simulink model "TorqueTest"  (R2026a)
settings: Solver=FixedStepAuto  StopTime=15  FixedStep=0.001  MinStep=1e-4
model workspace (MATLAB code in the model file):
  | K_d_1 = 0;
  | omegaFilter = 100;
  | 
  | 
  | % Motor parmeters
  | Km = 0.5;
  | 
  | % Gear ratio
  | i = 20;
  | 
  | %
  | IMax = 16;
  | IMin = - IMax;
undefined symbols (not defined in the file or in its folder): X, Y, Z
libraries: sm_lib x26, nesl_utility x16, slpidlib x1
settings Model: Creator=Bruker  LastModifiedBy=Bruker

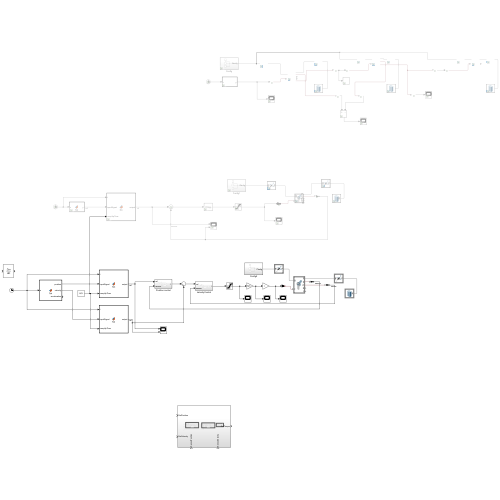
[thumbnail: Simulink's stored preview of the top-level diagram]
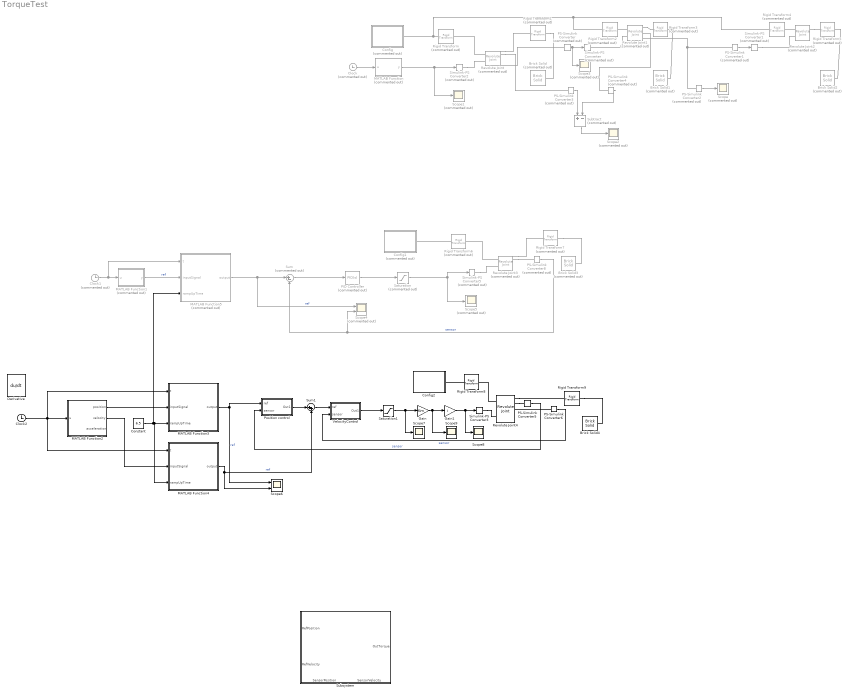
== system TorqueTest ==
  Brick Solid{,1..3} (4 alike) : sm_lib/Body Elements/Brick Solid  Commented=on  BrickDimensions=[1 0.1 0.1]  BrickDimensionsUnits=m  ExportEntireGeometry=off  InertiaType=CalculateFromGeometry  BasedOnType=Density  Density=1000  DensityUnits=kg/m^3  Mass=1  MassUnits=kg  CenterOfMass=[0 0 0]  CenterOfMassUnits=m  MomentsOfInertia=[1 1 1]  MomentsOfInertiaUnits=kg*m^2  ProductsOfInertia=[0 0 0]  ProductsOfInertiaUnits=kg*m^2  GraphicType=FromGeometry  MarkerShape=Sphere  MarkerSize=10  GraphicVisPropType=SimpleVisualProperties  GraphicDiffuseColor=[0.5 0.5 0.5]  GraphicOpacity=1  GraphicSpecularColor=[0.5 0.5 0.5 1.0]  GraphicAmbientColor=[0.15 0.15 0.15 1.0]  GraphicEmissiveColor=[0.0 0.0 0.0 1.0]  GraphicShininess=75  DoExposeReferenceFrame=on  SerializedFrames=<Frames/>
  Brick Solid4 : sm_lib/Body Elements/Brick Solid  BrickDimensions=[1 0.1 0.1]  BrickDimensionsUnits=m  ExportEntireGeometry=off  InertiaType=CalculateFromGeometry  BasedOnType=Density  Density=1000  DensityUnits=kg/m^3  Mass=1  MassUnits=kg  CenterOfMass=[0 0 0]  CenterOfMassUnits=m  MomentsOfInertia=[1 1 1]  MomentsOfInertiaUnits=kg*m^2  ProductsOfInertia=[0 0 0]  ProductsOfInertiaUnits=kg*m^2  GraphicType=FromGeometry  MarkerShape=Sphere  MarkerSize=10  GraphicVisPropType=SimpleVisualProperties  GraphicDiffuseColor=[0 0.3333 1]  GraphicOpacity=1  GraphicSpecularColor=[0.5 0.5 0.5 1.0]  GraphicAmbientColor=[0.15 0.15 0.15 1.0]  GraphicEmissiveColor=[0.0 0.0 0.0 1.0]  GraphicShininess=75  DoExposeReferenceFrame=on  SerializedFrames=<Frames/>
  Clock : Clock  Commented=on
  Clock1 : Clock  Commented=on
  Clock2 : Clock
  Config : Subsystem  Commented=on
  Config1 : Subsystem  Commented=on
  Config2 : Subsystem
  Constant : Constant  Value=6.5
  Derivative : Derivative
  Gain : Gain  Gain=Km
  Gain1 : Gain  Gain=i
  MATLAB Function : MATLAB Function  Commented=on  TreatAsAtomicUnit=on
  MATLAB Function1 : MATLAB Function  Commented=on  TreatAsAtomicUnit=on
  MATLAB Function2 : MATLAB Function  TreatAsAtomicUnit=on
  MATLAB Function3 : MATLAB Function  TreatAsAtomicUnit=on
  MATLAB Function4 : MATLAB Function  TreatAsAtomicUnit=on
  MATLAB Function5 : MATLAB Function  Commented=on  TreatAsAtomicUnit=on
  PID Controller : slpidlib/PID Controller  Commented=on  Controller=PID  Form=Parallel  TimeDomain=Continuous-time  UseExternalTs=off  SampleTime=-1  IntegratorMethod=Forward Euler  FilterMethod=Forward Euler  ControllerParametersSource=internal  P=750  I=0  UseKiTs=off  D=10  UseExternalDerivativeSource=off  N=100  UseFilter=on  TunerSelectOption=Transfer Function Based (PID Tuner App)  InitialConditionSource=internal  InitialConditionForIntegrator=0  InitialConditionForFilter=0  DifferentiatorICPrevScaledInput=0  ExternalReset=none  TrackingMode=off  Kt=1  LimitOutput=off  SatLimitsSource=internal  UpperSaturationLimit=inf  LowerSaturationLimit=-inf  LinearizeAsGain=on  AntiWindupMode=none  Kb=1  LimitIntegrator=off  UpperIntegratorSaturationLimit=inf  LowerIntegratorSaturationLimit=-inf  POutMin=[]  POutMax=[]  IOutMin=[]  IOutMax=[]  DOutMin=[]  DOutMax=[]  NOutMin=[]  NOutMax=[]  SumOutMin=[]  SumOutMax=[]  SaturationOutMin=[]  SaturationOutMax=[]  PParamMin=[]  PParamMax=[]  IParamMin=[]  IParamMax=[]  DParamMin=[]  DParamMax=[]  NParamMin=[]  NParamMax=[]  KbParamMin=[]  KbParamMax=[]  KtParamMin=[]  KtParamMax=[]  KbOutMin=[]  KbOutMax=[]  KtOutMin=[]  KtOutMax=[]  IntegratorOutMin=[]  IntegratorOutMax=[]  FilterOutMin=[]  FilterOutMax=[]  SumI1OutMin=[]  SumI1OutMax=[]  SumI2OutMin=[]  SumI2OutMax=[]  SumI3OutMin=[]  SumI3OutMax=[]  SumI4OutMin=[]  SumI4OutMax=[]  SumDOutMin=[]  SumDOutMax=[]  DifferentiatorOutMin=[]  DifferentiatorOutMax=[]  FilterDiffOutCoefMin=[]  FilterDiffOutCoefMax=[]  ReciprocalOutMin=[]  ReciprocalOutMax=[]  SumDenOutMin=[]  SumDenOutMax=[]  SumNumOutMin=[]  SumNumOutMax=[]  DivideOutMin=[]  DivideOutMax=[]  UdiffTsProdOutMin=[]  UdiffTsProdOutMax=[]  NTsProdOutMin=[]  NTsProdOutMax=[]  UintegralTsProdOutMin=[]  UintegralTsProdOutMax=[]  UngainTsProdOutMin=[]  UngainTsProdOutMax=[]  ClampingZeroOutDataTypeStr=Inherit: Inherit via back propagation  ClampingZeroOutMin=[]  ClampingZeroOutMax=[]  FilterDenConstantOutDataTypeStr=Inherit: Inherit via back propagation  FilterDenConstantOutMin=[]  FilterDenConstantOutMax=[]  PCopyOutDataTypeStr=Inherit: Inherit via back propagation  PCopyOutMin=[]  PCopyOutMax=[]  NCopyOutDataTypeStr=Inherit: Inherit via back propagation  NCopyOutMin=[]  NCopyOutMax=[]  IntegratorContinuousStateAttributes=''  IntegratorStateMustResolveToSignalObject=off  IntegratorRTWStateStorageClass=Auto  FilterContinuousStateAttributes=''  FilterStateMustResolveToSignalObject=off  FilterRTWStateStorageClass=Auto  ParallelPVariant=InternalParameters  IdealPVariant=Disabled  IVariant=InternalParameters  DVariant=InternalParameters  IntegratorVariant=Continuous  SatVariant=Disabled  AWVariant=Passthrough  PCopyVariant=Disabled  TRVariant=Disabled  FdbkBlocksVariant=Forward  IdealPFdbkVariant=Disabled  SatFdbkVariant=Disabled  DerivativeFilterVariant=ContFilter  NVariant=InternalParameters  NCopyVariant=Disabled  FilterICVariant=InternalICsFilter  IntegratorICVariant=InternalICs  ExternalResetVariant=Disabled  TRSumVariant=Passthrough  SumFdbkVariant=Disabled  SumVariant=Sum_PID  TsampFilterVariant=InternalTs  TsampNgainVariant=Passthrough  TsampIntegralVariant=Disabled_SignalSpec  ExternalSaturationOutDataTypeStr=Inherit: Same as second input  DerivativeSourceVariant=ErrorSignal  PreIntVariant=InternalPreInt
  PS-Simulink Converter{,1..4,8} (6 alike) : nesl_utility/PS-Simulink Converter  Commented=on  PhysicalDomain=network_engine_domain  SubClassName=ps_output  LeftPortType=input  RightPortType=output  PseudoPeriodic=off  Frequencies=[]  VectorFormat=inherit  Unit=inherit  AffineConversion=off
  PS-Simulink Converter5 : nesl_utility/PS-Simulink Converter  PhysicalDomain=network_engine_domain  SubClassName=ps_output  LeftPortType=input  RightPortType=output  PseudoPeriodic=off  Frequencies=[]  VectorFormat=inherit  Unit=inherit  AffineConversion=off
  PS-Simulink Converter6 : nesl_utility/PS-Simulink Converter  PhysicalDomain=network_engine_domain  SubClassName=ps_output  LeftPortType=input  RightPortType=output  PseudoPeriodic=off  Frequencies=[]  VectorFormat=inherit  Unit=inherit  AffineConversion=off
  Position control : Subsystem
  Revolute Joint : sm_lib/Joints/Revolute Joint  Commented=on  JointMode=Normal  CompositeWrenchDir=FollowerOnBase  CompositeWrenchFrame=BaseFrame  SenseConstraintForce=off  SenseConstraintTorque=off  SenseTotalForce=off  SenseTotalTorque=off  PositionTargetSpecify=off  PositionTargetPriority=Low  PositionTargetValue=0  PositionTargetValueUnits=deg  VelocityTargetSpecify=off  VelocityTargetPriority=High  VelocityTargetValue=0  VelocityTargetValueUnits=deg/s  EquilibriumPosition=0  EquilibriumPositionUnits=deg  SpringStiffness=0  SpringStiffnessUnits=N*m/deg  DampingCoefficient=0  DampingCoefficientUnits=N*m/(deg/s)  LowerLimitSpecify=off  LowerLimitBound=-90  LowerLimitBoundUnits=deg  LowerLimitStiffness=1e4  LowerLimitStiffnessUnits=N*m/deg  LowerLimitDamping=10  LowerLimitDampingUnits=N*m/(deg/s)  LowerLimitTransitionRegionWidth=0.1  LowerLimitTransitionRegionWidthUnits=deg  UpperLimitSpecify=off  UpperLimitBound=90  UpperLimitBoundUnits=deg  UpperLimitStiffness=1e4  UpperLimitStiffnessUnits=N*m/deg  UpperLimitDamping=10  UpperLimitDampingUnits=N*m/(deg/s)  UpperLimitTransitionRegionWidth=0.1  UpperLimitTransitionRegionWidthUnits=deg  TorqueActuationMode=ComputedTorque  MotionActuationMode=InputMotion  SensePosition=on  SenseVelocity=on  SenseAcceleration=on  SenseTorqueForce=on  SenseLowerLimitTorqueForce=off  SenseUpperLimitTorqueForce=off
  Revolute Joint1 : sm_lib/Joints/Revolute Joint  Commented=on  JointMode=Normal  CompositeWrenchDir=FollowerOnBase  CompositeWrenchFrame=BaseFrame  SenseConstraintForce=off  SenseConstraintTorque=off  SenseTotalForce=off  SenseTotalTorque=off  PositionTargetSpecify=off  PositionTargetPriority=High  PositionTargetValue=0  PositionTargetValueUnits=deg  VelocityTargetSpecify=off  VelocityTargetPriority=High  VelocityTargetValue=0  VelocityTargetValueUnits=deg/s  EquilibriumPosition=0  EquilibriumPositionUnits=deg  SpringStiffness=0  SpringStiffnessUnits=N*m/deg  DampingCoefficient=0  DampingCoefficientUnits=N*m/(deg/s)  LowerLimitSpecify=off  LowerLimitBound=-90  LowerLimitBoundUnits=deg  LowerLimitStiffness=1e4  LowerLimitStiffnessUnits=N*m/deg  LowerLimitDamping=10  LowerLimitDampingUnits=N*m/(deg/s)  LowerLimitTransitionRegionWidth=0.1  LowerLimitTransitionRegionWidthUnits=deg  UpperLimitSpecify=off  UpperLimitBound=90  UpperLimitBoundUnits=deg  UpperLimitStiffness=1e4  UpperLimitStiffnessUnits=N*m/deg  UpperLimitDamping=10  UpperLimitDampingUnits=N*m/(deg/s)  UpperLimitTransitionRegionWidth=0.1  UpperLimitTransitionRegionWidthUnits=deg  TorqueActuationMode=InputTorque  MotionActuationMode=ComputedMotion  SensePosition=on  SenseVelocity=off  SenseAcceleration=off  SenseTorqueForce=on  SenseLowerLimitTorqueForce=off  SenseUpperLimitTorqueForce=off
  Revolute Joint2 : sm_lib/Joints/Revolute Joint  Commented=on  JointMode=Normal  CompositeWrenchDir=FollowerOnBase  CompositeWrenchFrame=BaseFrame  SenseConstraintForce=off  SenseConstraintTorque=off  SenseTotalForce=off  SenseTotalTorque=off  PositionTargetSpecify=off  PositionTargetPriority=High  PositionTargetValue=0  PositionTargetValueUnits=deg  VelocityTargetSpecify=off  VelocityTargetPriority=High  VelocityTargetValue=0  VelocityTargetValueUnits=deg/s  EquilibriumPosition=0  EquilibriumPositionUnits=deg  SpringStiffness=0  SpringStiffnessUnits=N*m/deg  DampingCoefficient=0  DampingCoefficientUnits=N*m/(deg/s)  LowerLimitSpecify=off  LowerLimitBound=-90  LowerLimitBoundUnits=deg  LowerLimitStiffness=1e4  LowerLimitStiffnessUnits=N*m/deg  LowerLimitDamping=10  LowerLimitDampingUnits=N*m/(deg/s)  LowerLimitTransitionRegionWidth=0.1  LowerLimitTransitionRegionWidthUnits=deg  UpperLimitSpecify=off  UpperLimitBound=90  UpperLimitBoundUnits=deg  UpperLimitStiffness=1e4  UpperLimitStiffnessUnits=N*m/deg  UpperLimitDamping=10  UpperLimitDampingUnits=N*m/(deg/s)  UpperLimitTransitionRegionWidth=0.1  UpperLimitTransitionRegionWidthUnits=deg  TorqueActuationMode=InputTorque  MotionActuationMode=ComputedMotion  SensePosition=off  SenseVelocity=off  SenseAcceleration=off  SenseTorqueForce=on  SenseLowerLimitTorqueForce=off  SenseUpperLimitTorqueForce=off
  Revolute Joint3 : sm_lib/Joints/Revolute Joint  Commented=on  JointMode=Normal  CompositeWrenchDir=FollowerOnBase  CompositeWrenchFrame=BaseFrame  SenseConstraintForce=off  SenseConstraintTorque=off  SenseTotalForce=off  SenseTotalTorque=off  PositionTargetSpecify=off  PositionTargetPriority=Low  PositionTargetValue=0  PositionTargetValueUnits=deg  VelocityTargetSpecify=off  VelocityTargetPriority=High  VelocityTargetValue=0  VelocityTargetValueUnits=deg/s  EquilibriumPosition=0  EquilibriumPositionUnits=deg  SpringStiffness=0  SpringStiffnessUnits=N*m/deg  DampingCoefficient=0  DampingCoefficientUnits=N*m/(deg/s)  LowerLimitSpecify=off  LowerLimitBound=-90  LowerLimitBoundUnits=deg  LowerLimitStiffness=1e4  LowerLimitStiffnessUnits=N*m/deg  LowerLimitDamping=10  LowerLimitDampingUnits=N*m/(deg/s)  LowerLimitTransitionRegionWidth=0.1  LowerLimitTransitionRegionWidthUnits=deg  UpperLimitSpecify=off  UpperLimitBound=90  UpperLimitBoundUnits=deg  UpperLimitStiffness=1e4  UpperLimitStiffnessUnits=N*m/deg  UpperLimitDamping=10  UpperLimitDampingUnits=N*m/(deg/s)  UpperLimitTransitionRegionWidth=0.1  UpperLimitTransitionRegionWidthUnits=deg  TorqueActuationMode=InputTorque  MotionActuationMode=ComputedMotion  SensePosition=on  SenseVelocity=on  SenseAcceleration=on  SenseTorqueForce=on  SenseLowerLimitTorqueForce=off  SenseUpperLimitTorqueForce=off
  Revolute Joint4 : sm_lib/Joints/Revolute Joint  JointMode=Normal  CompositeWrenchDir=FollowerOnBase  CompositeWrenchFrame=BaseFrame  SenseConstraintForce=off  SenseConstraintTorque=off  SenseTotalForce=off  SenseTotalTorque=off  PositionTargetSpecify=off  PositionTargetPriority=Low  PositionTargetValue=0  PositionTargetValueUnits=deg  VelocityTargetSpecify=off  VelocityTargetPriority=High  VelocityTargetValue=0  VelocityTargetValueUnits=deg/s  EquilibriumPosition=0  EquilibriumPositionUnits=deg  SpringStiffness=0  SpringStiffnessUnits=N*m/deg  DampingCoefficient=0  DampingCoefficientUnits=N*m/(deg/s)  LowerLimitSpecify=off  LowerLimitBound=-90  LowerLimitBoundUnits=deg  LowerLimitStiffness=1e4  LowerLimitStiffnessUnits=N*m/deg  LowerLimitDamping=10  LowerLimitDampingUnits=N*m/(deg/s)  LowerLimitTransitionRegionWidth=0.1  LowerLimitTransitionRegionWidthUnits=deg  UpperLimitSpecify=off  UpperLimitBound=90  UpperLimitBoundUnits=deg  UpperLimitStiffness=1e4  UpperLimitStiffnessUnits=N*m/deg  UpperLimitDamping=10  UpperLimitDampingUnits=N*m/(deg/s)  UpperLimitTransitionRegionWidth=0.1  UpperLimitTransitionRegionWidthUnits=deg  TorqueActuationMode=InputTorque  MotionActuationMode=ComputedMotion  SensePosition=on  SenseVelocity=on  SenseAcceleration=on  SenseTorqueForce=on  SenseLowerLimitTorqueForce=off  SenseUpperLimitTorqueForce=off
  Rigid Transform{,2,4,6} (4 alike) : sm_lib/Frames and Transforms/Rigid Transform  Commented=on  RotationMethod=RotationSequence  FollAlignAxisA=+X  BaseAlignAxisA=+Y  FollAlignAxisB=+Y  BaseAlignAxisB=+Z  RotationStandardAxis=+Z  RotationAngle=0  RotationAngleUnits=deg  RotationArbitraryAxis=[0 0 1]  RotationSequenceAxes=FollowerAxes  RotationSequence=XYX  RotationSequenceAngles=[90 0 0]  RotationSequenceAnglesUnits=deg  RotationMatrix=[1 0 0;0 1 0;0 0 1]  Quaternion=[1 0 0 0]  TranslationMethod=None  TranslationCartesianOffset=[0 0 0]  TranslationCartesianOffsetUnits=m  TranslationStandardAxis=+Z  TranslationStandardOffset=0  TranslationStandardOffsetUnits=m  TranslationROffset=0  TranslationROffsetUnits=m  TranslationThetaOffset=0  TranslationThetaOffsetUnits=deg  TranslationZOffset=0  TranslationZOffsetUnits=m
  Rigid Transform{1,3,5,7} (4 alike) : sm_lib/Frames and Transforms/Rigid Transform  Commented=on  RotationMethod=RotationSequence  FollAlignAxisA=+X  BaseAlignAxisA=+Y  FollAlignAxisB=+Y  BaseAlignAxisB=+Z  RotationStandardAxis=+Z  RotationAngle=0  RotationAngleUnits=deg  RotationArbitraryAxis=[0 0 1]  RotationSequenceAxes=FollowerAxes  RotationSequence=XYX  RotationSequenceAngles=[90 0 0]  RotationSequenceAnglesUnits=deg  RotationMatrix=[1 0 0;0 1 0;0 0 1]  Quaternion=[1 0 0 0]  TranslationMethod=Cartesian  TranslationCartesianOffset=[0.5 0 0]  TranslationCartesianOffsetUnits=m  TranslationStandardAxis=+Z  TranslationStandardOffset=0  TranslationStandardOffsetUnits=m  TranslationROffset=0  TranslationROffsetUnits=m  TranslationThetaOffset=0  TranslationThetaOffsetUnits=deg  TranslationZOffset=0  TranslationZOffsetUnits=m
  Rigid Transform8 : sm_lib/Frames and Transforms/Rigid Transform  RotationMethod=RotationSequence  FollAlignAxisA=+X  BaseAlignAxisA=+Y  FollAlignAxisB=+Y  BaseAlignAxisB=+Z  RotationStandardAxis=+Z  RotationAngle=0  RotationAngleUnits=deg  RotationArbitraryAxis=[0 0 1]  RotationSequenceAxes=FollowerAxes  RotationSequence=XYX  RotationSequenceAngles=[90 0 0]  RotationSequenceAnglesUnits=deg  RotationMatrix=[1 0 0;0 1 0;0 0 1]  Quaternion=[1 0 0 0]  TranslationMethod=None  TranslationCartesianOffset=[0 0 0]  TranslationCartesianOffsetUnits=m  TranslationStandardAxis=+Z  TranslationStandardOffset=0  TranslationStandardOffsetUnits=m  TranslationROffset=0  TranslationROffsetUnits=m  TranslationThetaOffset=0  TranslationThetaOffsetUnits=deg  TranslationZOffset=0  TranslationZOffsetUnits=m
  Rigid Transform9 : sm_lib/Frames and Transforms/Rigid Transform  RotationMethod=RotationSequence  FollAlignAxisA=+X  BaseAlignAxisA=+Y  FollAlignAxisB=+Y  BaseAlignAxisB=+Z  RotationStandardAxis=+Z  RotationAngle=0  RotationAngleUnits=deg  RotationArbitraryAxis=[0 0 1]  RotationSequenceAxes=FollowerAxes  RotationSequence=XYX  RotationSequenceAngles=[90 0 0]  RotationSequenceAnglesUnits=deg  RotationMatrix=[1 0 0;0 1 0;0 0 1]  Quaternion=[1 0 0 0]  TranslationMethod=Cartesian  TranslationCartesianOffset=[0.5 0 0]  TranslationCartesianOffsetUnits=m  TranslationStandardAxis=+Z  TranslationStandardOffset=0  TranslationStandardOffsetUnits=m  TranslationROffset=0  TranslationROffsetUnits=m  TranslationThetaOffset=0  TranslationThetaOffsetUnits=deg  TranslationZOffset=0  TranslationZOffsetUnits=m
  Saturation : Saturate  Commented=on  UpperLimit=200  LowerLimit=-200
  Saturation1 : Saturate  UpperLimit=IMax  LowerLimit=IMin
  Scope{,1..3,5} (5 alike) : Scope  Commented=on
      Scope settings: ActiveDisplayYMinimum=-352.45894049159494  ActiveDisplayYMaximum=1009.6712365398308
      Scope1 settings: ActiveDisplayYMinimum=-1  ActiveDisplayYMaximum=1
      Scope2 settings: ActiveDisplayYMinimum=-60.70451241279882  ActiveDisplayYMaximum=48.625230918631289  DataLoggingVariableName=ScopeData2
      Scope3 settings: ActiveDisplayYMinimum=-165.73958307555844  ActiveDisplayYMaximum=1001.1562497821226  DataLoggingVariableName=ScopeData3
      Scope5 settings: ActiveDisplayYMinimum=-1  ActiveDisplayYMaximum=1  DataLoggingVariableName=ScopeData5
  Scope4 : Scope  Commented=on  NumInputPorts=2
      settings: ActiveDisplayYMinimum=-10.0433259629833  ActiveDisplayYMaximum=10.142230414759299  DataLoggingVariableName=ScopeData4
  Scope6 : Scope  NumInputPorts=2
      settings: ActiveDisplayYMinimum=4.5607316054471223  ActiveDisplayYMaximum=7.6819973674434889  DataLoggingVariableName=ScopeData8
  Scope7 : Scope
      settings: ActiveDisplayYMinimum=-1  ActiveDisplayYMaximum=1  DataLoggingVariableName=ScopeData9
  Scope8 : Scope
      settings: ActiveDisplayYMinimum=-188.78487408116746  ActiveDisplayYMaximum=99.063866730507073  DataLoggingVariableName=ScopeData10
  Scope9 : Scope
      settings: DataLoggingVariableName=ScopeData11
  Simulink-PS Converter{,1..2,5} (4 alike) : nesl_utility/Simulink-PS Converter  Commented=on  PhysicalDomain=network_engine_domain  SubClassName=ps_input  LeftPortType=input  RightPortType=output  PseudoPeriodic=off  Frequencies=[]  NoiseDistribution=none  NoiseParameters=[]  Unit=1  AffineConversion=off  FilteringAndDerivatives=filter  SimscapeFilterOrder=2  InputFilterTimeConstant=0.001  UdotUserProvided=0
  Simulink-PS Converter3 : nesl_utility/Simulink-PS Converter  PhysicalDomain=network_engine_domain  SubClassName=ps_input  LeftPortType=input  RightPortType=output  PseudoPeriodic=off  Frequencies=[]  NoiseDistribution=none  NoiseParameters=[]  Unit=1  AffineConversion=off  FilteringAndDerivatives=provide  SimscapeFilterOrder=1  InputFilterTimeConstant=0.001  UdotUserProvided=0
  Subsystem : Subsystem
      settings: PortSchema="{\"entries\":[{\"content\":{\"sides\":[{\"content\":{\"connectorIds\":[\"In1\",\"In2\"]},\"type\":\"ConnectorPlacement.EquallySpacedRectSide\",\"uuid\":\"51550f40-279e-4723-9a78-98dcf3f698a2\"},{\"content\":{\"connectorIds\":[\"Out1\"],\"side\":\"RIGHT\"},\"type\":\"ConnectorPlacement.EquallySpacedRectSide\",\"uuid\":\"f243d76f-4e9d-407e-a230-76bea4453255\"},{\"content\":{\"side\":\"TOP\"},\"type\":\"ConnectorPlacement.EquallySpacedRectSide\",\"uuid\":\"5b6b6dd7-8a33-494a-8ee5-fc7698c2bf83\"},{\"content\":{\"connectorIds\":[\"In3\",\"In4\"],\"side\":\"BOTTOM\"},\"type\":\"ConnectorPlacement.EquallySpacedRectSide\",\"uuid\":\"d720744c-358d-4588-a5fe-fa324fd98b41\"}]},\"type\":\"ConnectorPlacement.EquallySpacedConnector\",\"uuid\":\"b5ef8a6e-2b84-4a51-bcfc-62a4469380e6\"}],\"packageUris\":[\"http://schema.mathworks.com/mf0/Connector/R2020b\"],\"version\":\"1.0\"}"
  Subtract : Sum  Commented=on  Inputs=+-
  Sum : Sum  Commented=on  Inputs=|+-
  Sum1 : Sum  Inputs=|++
  VelocityControl : Subsystem
  wires:
  PS-Simulink Converter/1 -> Scope3/1, Simulink-PS Converter/1
  PS-Simulink Converter1/1 -> Simulink-PS Converter1/1
  PS-Simulink Converter2/1 -> Scope/1
  Clock/1 -> MATLAB Function/1(u)
  MATLAB Function/1(y) -> Scope1/1, Simulink-PS Converter2/1
  PS-Simulink Converter3/1 -> Subtract/1
  PS-Simulink Converter4/1 -> Subtract/2
  Subtract/1 -> Scope2/1
  Clock1/1 -> MATLAB Function5/1(t), MATLAB Function1/1(u)
  PID Controller/1 -> Saturation/1
  PS-Simulink Converter8/1 -> Scope4/2, Sum/2  "sensor"
  Sum/1 -> PID Controller/1
  Saturation/1 -> Simulink-PS Converter5/1, Scope5/1
  Clock2/1 -> MATLAB Function3/1(t), MATLAB Function2/1(u), MATLAB Function4/1(t)
  MATLAB Function2/1(position) -> MATLAB Function3/2(inputSignal)
  Constant/1 -> MATLAB Function5/3(rampUpTime), MATLAB Function4/3(rampUpTime), MATLAB Function3/3(rampUpTime)
  MATLAB Function2/2(velocity) -> MATLAB Function4/2(inputSignal)
  MATLAB Function3/1(output) -> Scope6/1, Position control/1(ref)  "ref"
  MATLAB Function4/1(output) -> Sum1/2, Scope6/2  "ref"
  Gain1/1 -> Scope8/1, Simulink-PS Converter3/1
  Saturation1/1 -> Scope7/1, Gain/1
  Gain/1 -> Scope9/1, Gain1/1
  MATLAB Function1/1(y) -> MATLAB Function5/2(inputSignal)  "ref"
  MATLAB Function5/1(output) -> Scope4/1, Sum/1  "ref"
  VelocityControl/1(Out1) -> Saturation1/1
  PS-Simulink Converter5/1 -> Position control/2(sensor)  "sensor"
  PS-Simulink Converter6/1 -> VelocityControl/2(sensor)  "sensor"
  Sum1/1 -> VelocityControl/1(ref)
  Position control/1(Out1) -> Sum1/1
  connections:
  Revolute Joint/LConn1 -- Rigid Transform/RConn1
  Rigid Transform/LConn1 -- Rigid Transform2/LConn1 -- Rigid Transform4/LConn1 -- Config/RConn1
  Revolute Joint/RConn1 -- Rigid Transform1/LConn1
  Rigid Transform1/RConn1 -- Brick Solid/RConn1
  Revolute Joint1/RConn1 -- Rigid Transform3/LConn1
  Revolute Joint1/LConn1 -- Rigid Transform2/RConn1
  Rigid Transform3/RConn1 -- Brick Solid1/RConn1
  PS-Simulink Converter/LConn1 -- Revolute Joint/RConn5
  Revolute Joint1/LConn2 -- Simulink-PS Converter/RConn1
  Revolute Joint2/LConn1 -- Rigid Transform4/RConn1
  Revolute Joint2/RConn1 -- Rigid Transform5/LConn1
  Rigid Transform5/RConn1 -- Brick Solid2/RConn1
  Simulink-PS Converter1/RConn1 -- Revolute Joint2/LConn2
  PS-Simulink Converter1/LConn1 -- PS-Simulink Converter2/LConn1 -- Revolute Joint1/RConn3
  Simulink-PS Converter2/RConn1 -- Revolute Joint/LConn2
  Revolute Joint/RConn2 -- PS-Simulink Converter3/LConn1
  PS-Simulink Converter4/LConn1 -- Revolute Joint1/RConn2
  Rigid Transform6/LConn1 -- Config1/RConn1
  Simulink-PS Converter5/RConn1 -- Revolute Joint3/LConn2
  Revolute Joint3/RConn2 -- PS-Simulink Converter8/LConn1
  Rigid Transform7/RConn1 -- Brick Solid3/RConn1
  Revolute Joint3/RConn1 -- Rigid Transform7/LConn1
  Revolute Joint3/LConn1 -- Rigid Transform6/RConn1
  Revolute Joint4/LConn1 -- Rigid Transform8/RConn1
  Rigid Transform8/LConn1 -- Config2/RConn1
  Revolute Joint4/RConn1 -- Rigid Transform9/LConn1
  Revolute Joint4/RConn2 -- PS-Simulink Converter5/LConn1
  Rigid Transform9/RConn1 -- Brick Solid4/RConn1
  PS-Simulink Converter6/LConn1 -- Revolute Joint4/RConn3
  Simulink-PS Converter3/RConn1 -- Revolute Joint4/LConn2

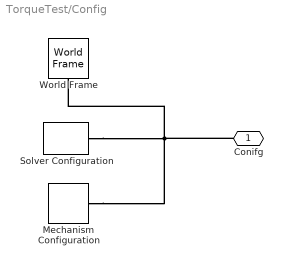
== system TorqueTest/Config ==
  Mechanism Configuration : sm_lib/Utilities/Mechanism Configuration  UniformGravity=Constant  GravityVector=[0 0 -9.81]  GravityVectorUnits=m/s^2  LinearizationDelta=0.001  JointModeTransitionNonlinearIterations=2
  Solver Configuration : nesl_utility/Solver Configuration  PhysicalDomain=network_engine_domain  SubClassName=solver  LeftPortType=input  RightPortType=generic  Tones=[]  Harmonics=[]  SimulateNoise=off  Profile=off  UseLocalSampling=off  EnableSwitchedLinearOptims=on  FrequencyDomain=off  UseCCode=off  RelTol=0.001  AbsTol=1e-06  MinStep=1e-09  ToWorkspace=off  RevertToSquareIcSolve=off  NumHomotopyIterations=100  PhasorMode=off  PhasorModeNumHarmonics=1  ConsistencySolver=NEWTON_FTOL  CanonicalOrdering=UNORDERED  OptimizeIntermediates=UNOPTIMIZED  IndexReductionMethod=DerivativeReplacement  DoDC=off  ResidualTolerance=1e-9  ConsistencyTolSource=GLOBAL  ConsistencyAbsTol=0.001  ConsistencyRelTol=0.001  ConsistencyTolFactor=0.001  UseLocalSolver=off  LocalSolverChoice=NE_BACKWARD_EULER_ADVANCER  ResolveIndetEquations=on  FunctionEvalNumThread=1  LocalSolverSampleTime=.001  DoFixedCost=off  MaxNonlinIter=3  MaxModeIter=2  ComputeImpulses=off  ImpulseIterations=2  LinearAlgebra=Sparse  LinearAlgebraNumThread=0  EquationFormulation=NE_TIME_EF  DelaysMemoryBudget=1024  AutomaticFiltering=on  FilteringTimeConstant=0.001  PartitionStorageMethod=AS_NEEDED  PartitionMemoryBudget=1024  PartitionMethod=FAST  MultibodyUseLocalSolver=off  MultibodyLocalSolverChoice=ODE1  MultibodyLocalSolverSampleTime=0.001
  World Frame : sm_lib/Frames and Transforms/World Frame
  Conifg : PMIOPort  Side=Right
  connections:
  Solver Configuration/RConn1 -- Conifg/RConn1 -- Mechanism Configuration/RConn1 -- World Frame/RConn1

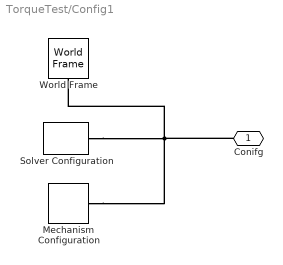
== system TorqueTest/Config1 ==
  Mechanism Configuration : sm_lib/Utilities/Mechanism Configuration  UniformGravity=Constant  GravityVector=[0 0 -9.81]  GravityVectorUnits=m/s^2  LinearizationDelta=0.001  JointModeTransitionNonlinearIterations=2
  Solver Configuration : nesl_utility/Solver Configuration  PhysicalDomain=network_engine_domain  SubClassName=solver  LeftPortType=input  RightPortType=generic  Tones=[]  Harmonics=[]  SimulateNoise=off  Profile=off  UseLocalSampling=off  EnableSwitchedLinearOptims=on  FrequencyDomain=off  UseCCode=off  RelTol=0.001  AbsTol=1e-06  MinStep=1e-09  ToWorkspace=off  RevertToSquareIcSolve=off  NumHomotopyIterations=100  PhasorMode=off  PhasorModeNumHarmonics=1  ConsistencySolver=NEWTON_FTOL  CanonicalOrdering=UNORDERED  OptimizeIntermediates=UNOPTIMIZED  IndexReductionMethod=DerivativeReplacement  DoDC=off  ResidualTolerance=1e-9  ConsistencyTolSource=GLOBAL  ConsistencyAbsTol=0.001  ConsistencyRelTol=0.001  ConsistencyTolFactor=0.001  UseLocalSolver=off  LocalSolverChoice=NE_BACKWARD_EULER_ADVANCER  ResolveIndetEquations=on  FunctionEvalNumThread=1  LocalSolverSampleTime=.001  DoFixedCost=off  MaxNonlinIter=3  MaxModeIter=2  ComputeImpulses=off  ImpulseIterations=2  LinearAlgebra=Sparse  LinearAlgebraNumThread=0  EquationFormulation=NE_TIME_EF  DelaysMemoryBudget=1024  AutomaticFiltering=on  FilteringTimeConstant=0.001  PartitionStorageMethod=AS_NEEDED  PartitionMemoryBudget=1024  PartitionMethod=FAST  MultibodyUseLocalSolver=off  MultibodyLocalSolverChoice=ODE1  MultibodyLocalSolverSampleTime=0.001
  World Frame : sm_lib/Frames and Transforms/World Frame
  Conifg : PMIOPort  Side=Right
  connections:
  Solver Configuration/RConn1 -- Conifg/RConn1 -- Mechanism Configuration/RConn1 -- World Frame/RConn1

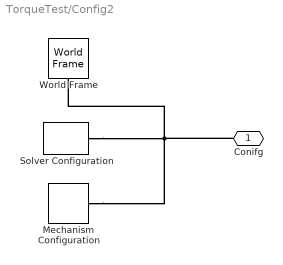
== system TorqueTest/Config2 ==
  Mechanism Configuration : sm_lib/Utilities/Mechanism Configuration  UniformGravity=Constant  GravityVector=[0 0 -9.81]  GravityVectorUnits=m/s^2  LinearizationDelta=0.001  JointModeTransitionNonlinearIterations=2
  Solver Configuration : nesl_utility/Solver Configuration  PhysicalDomain=network_engine_domain  SubClassName=solver  LeftPortType=input  RightPortType=generic  Tones=[]  Harmonics=[]  SimulateNoise=off  Profile=off  UseLocalSampling=off  EnableSwitchedLinearOptims=on  FrequencyDomain=off  UseCCode=off  RelTol=0.001  AbsTol=1e-06  MinStep=1e-09  ToWorkspace=off  RevertToSquareIcSolve=off  NumHomotopyIterations=100  PhasorMode=off  PhasorModeNumHarmonics=1  ConsistencySolver=NEWTON_FTOL  CanonicalOrdering=UNORDERED  OptimizeIntermediates=UNOPTIMIZED  IndexReductionMethod=DerivativeReplacement  DoDC=off  ResidualTolerance=1e-9  ConsistencyTolSource=GLOBAL  ConsistencyAbsTol=0.001  ConsistencyRelTol=0.001  ConsistencyTolFactor=0.001  UseLocalSolver=off  LocalSolverChoice=NE_BACKWARD_EULER_ADVANCER  ResolveIndetEquations=on  FunctionEvalNumThread=1  LocalSolverSampleTime=.001  DoFixedCost=off  MaxNonlinIter=3  MaxModeIter=2  ComputeImpulses=off  ImpulseIterations=2  LinearAlgebra=Sparse  LinearAlgebraNumThread=0  EquationFormulation=NE_TIME_EF  DelaysMemoryBudget=1024  AutomaticFiltering=on  FilteringTimeConstant=0.001  PartitionStorageMethod=AS_NEEDED  PartitionMemoryBudget=1024  PartitionMethod=FAST  MultibodyUseLocalSolver=off  MultibodyLocalSolverChoice=ODE1  MultibodyLocalSolverSampleTime=0.001
  World Frame : sm_lib/Frames and Transforms/World Frame
  Conifg : PMIOPort  Side=Right
  connections:
  Solver Configuration/RConn1 -- Conifg/RConn1 -- Mechanism Configuration/RConn1 -- World Frame/RConn1

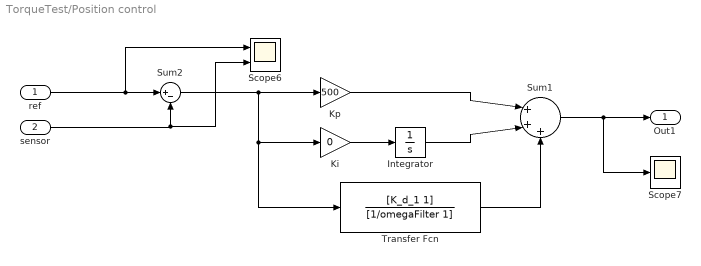
== system TorqueTest/Position control ==
  ref : Inport
  sensor : Inport  Port=2
  Integrator : Integrator
  Ki : Gain  Gain=0
  Kp : Gain  Gain=500
  Scope6 : Scope  NumInputPorts=2
      settings: ActiveDisplayYMinimum=2.0966055880111791  ActiveDisplayYMaximum=2.2901843246411744  DataLoggingVariableName=ScopeData6
  Scope7 : Scope
      settings: ActiveDisplayYMinimum=-8.0651623624508559  ActiveDisplayYMaximum=8.5043450071059734  DataLoggingVariableName=ScopeData7
  Sum1 : Sum  Inputs=|+++
  Sum2 : Sum  Inputs=|+-
  Transfer Fcn : TransferFcn  Numerator=[K_d_1 1]  Denominator=[1/omegaFilter 1]
  Out1 : Outport
  wires:
  sensor/1 -> Scope6/2, Sum2/2
  ref/1 -> Scope6/1, Sum2/1
  Ki/1 -> Integrator/1
  Integrator/1 -> Sum1/2
  Sum2/1 -> Kp/1, Transfer Fcn/1, Ki/1
  Kp/1 -> Sum1/1
  Sum1/1 -> Out1/1, Scope7/1
  Transfer Fcn/1 -> Sum1/3

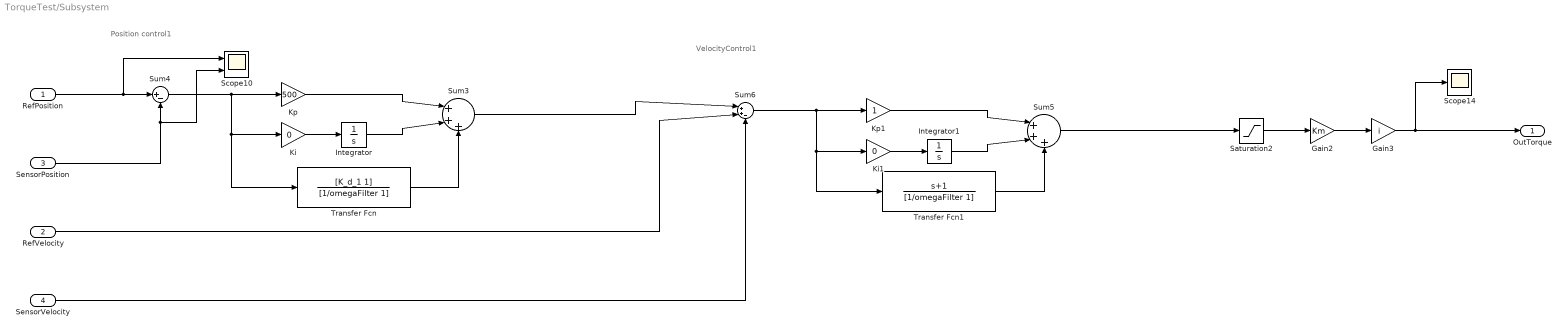
== system TorqueTest/Subsystem ==
  note: VelocityControl1
  note: Position control1
  RefPosition : Inport
  RefVelocity : Inport  Port=2
  SensorPosition : Inport  Port=3
  SensorVelocity : Inport  Port=4
  Gain2 : Gain  Gain=Km
  Gain3 : Gain  Gain=i
  Integrator : Integrator
  Integrator1 : Integrator
  Ki : Gain  Gain=0
  Ki1 : Gain  Gain=0
  Kp : Gain  Gain=500
  Kp1 : Gain
  Saturation2 : Saturate  UpperLimit=IMax  LowerLimit=IMin
  Scope10 : Scope  NumInputPorts=2
      settings: ActiveDisplayYMinimum=2.0966055880111791  ActiveDisplayYMaximum=2.2901843246411744  DataLoggingVariableName=ScopeData6
  Scope14 : Scope
      settings: DataLoggingVariableName=ScopeData12
  Sum3 : Sum  Inputs=|+++
  Sum4 : Sum  Inputs=|+-
  Sum5 : Sum  Inputs=|+++
  Sum6 : Sum  Inputs=|++-
  Transfer Fcn : TransferFcn  Numerator=[K_d_1 1]  Denominator=[1/omegaFilter 1]
  Transfer Fcn1 : TransferFcn  Numerator=[1 1]  Denominator=[1/omegaFilter 1]
  OutTorque : Outport
  wires:
  Gain2/1 -> Gain3/1
  Sum6/1 -> Kp1/1, Transfer Fcn1/1, Ki1/1
  Gain3/1 -> OutTorque/1, Scope14/1
  RefPosition/1 -> Scope10/1, Sum4/1
  Transfer Fcn/1 -> Sum3/3
  RefVelocity/1 -> Sum6/2
  SensorVelocity/1 -> Sum6/3
  Ki1/1 -> Integrator1/1
  Saturation2/1 -> Gain2/1
  SensorPosition/1 -> Scope10/2, Sum4/2
  Kp1/1 -> Sum5/1
  Sum3/1 -> Sum6/1
  Ki/1 -> Integrator/1
  Sum4/1 -> Kp/1, Transfer Fcn/1, Ki/1
  Integrator/1 -> Sum3/2
  Kp/1 -> Sum3/1
  Sum5/1 -> Saturation2/1
  Transfer Fcn1/1 -> Sum5/3
  Integrator1/1 -> Sum5/2

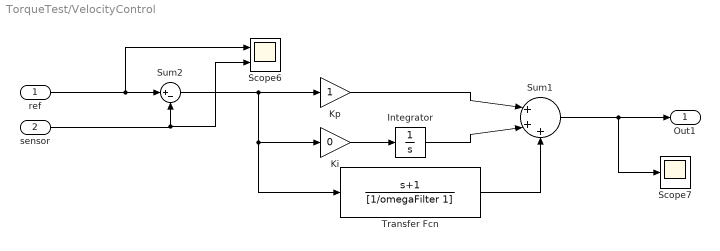
== system TorqueTest/VelocityControl ==
  ref : Inport
  sensor : Inport  Port=2
  Integrator : Integrator
  Ki : Gain  Gain=0
  Kp : Gain
  Scope6 : Scope  NumInputPorts=2
      settings: ActiveDisplayYMinimum=-11.217650017692428  ActiveDisplayYMaximum=11.569009438558426  DataLoggingVariableName=ScopeData6
  Scope7 : Scope
      settings: ActiveDisplayYMinimum=-18.650940091029479  ActiveDisplayYMaximum=25.667029395187896  DataLoggingVariableName=ScopeData7
  Sum1 : Sum  Inputs=|+++
  Sum2 : Sum  Inputs=|+-
  Transfer Fcn : TransferFcn  Numerator=[1 1]  Denominator=[1/omegaFilter 1]
  Out1 : Outport
  wires:
  sensor/1 -> Scope6/2, Sum2/2
  Transfer Fcn/1 -> Sum1/3
  ref/1 -> Scope6/1, Sum2/1
  Ki/1 -> Integrator/1
  Integrator/1 -> Sum1/2
  Sum1/1 -> Out1/1, Scope7/1
  Sum2/1 -> Kp/1, Transfer Fcn/1, Ki/1
  Kp/1 -> Sum1/1

== matlab function TorqueTest/MATLAB Function ==
  data: u input; y output
function y = fcn(u)

y = u/2;

== matlab function TorqueTest/MATLAB Function2 ==
  data: u input; position output; velocity output; acceleration output
function [position, velocity, acceleration] = fcn(u)

position = 8*sin(u);
velocity = 8*cos(u);
acceleration = -8*cos(u);

== matlab function TorqueTest/MATLAB Function3 ==
  data: t input; inputSignal input; output output; rampUpTime input
function output = fcn(t, inputSignal, rampUpTime)

if t < rampUpTime
    output = inputSignal * (t/rampUpTime);
else
    output = inputSignal;
end

== matlab function TorqueTest/MATLAB Function4 ==
  data: t input; inputSignal input; output output; rampUpTime input
function output = fcn(t, inputSignal, rampUpTime)

if t < rampUpTime
    output = inputSignal * (t/rampUpTime);
else
    output = inputSignal;
end

== matlab function TorqueTest/MATLAB Function5 ==
  data: t input; inputSignal input; output output; rampUpTime input
function output = fcn(t, inputSignal, rampUpTime)

if t < rampUpTime
    output = inputSignal * (t/rampUpTime);
else
    output = inputSignal;
end

== matlab function TorqueTest/MATLAB Function1 ==
  data: u input; y output
function y = fcn(u)

y = 8*sin(u);
